simulink model "guidebot_mil"  (R2024a)
settings: Solver=FixedStepDiscrete  StartTime=0  StopTime=60.0  FixedStep=0.05  RelTol=1e-3
InitFcn:
  | gb_setup_base();
undefined symbols (not defined in the file or in its folder): GB_X0
settings Model: Creator=asus  LastModifiedBy=asus

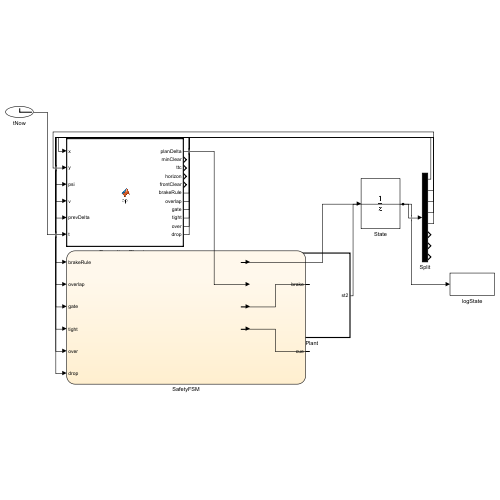
[thumbnail: Simulink's stored preview of the top-level diagram]
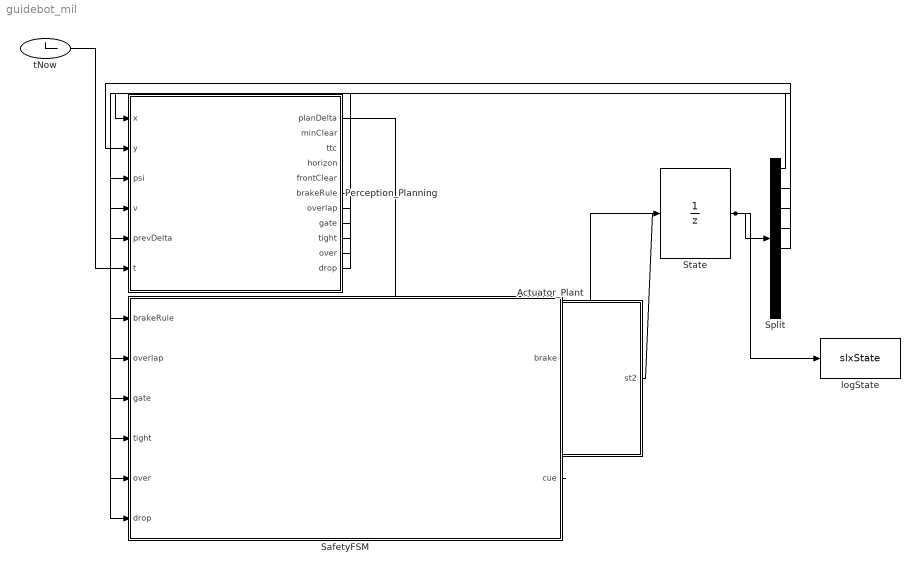
== system guidebot_mil ==
  Actuator_Plant : MATLAB Function  TreatAsAtomicUnit=on
  Perception_Planning : MATLAB Function  TreatAsAtomicUnit=on
  SafetyFSM : Stateflow chart  TreatAsAtomicUnit=on
  Split : Demux  Outputs=8
  State : UnitDelay  InitialCondition=GB_X0  SampleTime=0.05  HasFrameUpgradeWarning=on
  logState : ToWorkspace  VariableName=slxState  SaveFormat=Structure With Time  SampleTime=-1
  tNow : Clock
  wires:
  State/1 -> Split/1, Actuator_Plant/1(st), logState/1
  tNow/1 -> Perception_Planning/6(t)
  Split/1 -> Perception_Planning/1(x)
  Split/2 -> Perception_Planning/2(y)
  Split/3 -> Perception_Planning/3(psi)
  Split/4 -> Perception_Planning/4(v)
  Split/5 -> Perception_Planning/5(prevDelta)
  Perception_Planning/1(planDelta) -> Actuator_Plant/2(planDelta)
  Perception_Planning/6(brakeRule) -> SafetyFSM/1(brakeRule)
  Perception_Planning/7(overlap) -> SafetyFSM/2(overlap)
  Perception_Planning/8(gate) -> SafetyFSM/3(gate)
  Perception_Planning/9(tight) -> SafetyFSM/4(tight)
  Perception_Planning/10(over) -> SafetyFSM/5(over)
  Perception_Planning/11(drop) -> SafetyFSM/6(drop)
  SafetyFSM/1(brake) -> Actuator_Plant/3(brake)
  SafetyFSM/2(cue) -> Actuator_Plant/4(cue)
  Actuator_Plant/1(st2) -> State/1

== matlab function guidebot_mil/Actuator_Plant ==
  data: st input; st2 output; planDelta input; brake input; cue input
function st2 = ap(st,planDelta,brake,cue)
dt=0.050000; WB=0.450000; RR=0.220000; HW=2.000000;
pref=1.150000; slowF=0.500000; Tr=0.350000; slewDps=150.000000;
x=st(1); y=st(2); psi=st(3); v=st(4); prevDelta=st(5); tgt=st(6); bk=st(7); held=st(8);
maxStep=(slewDps*pi/180.0)*dt;
delta=planDelta; step=delta-prevDelta;
if step>maxStep, step=maxStep; end
if step<-maxStep, step=-maxStep; end
delta=prevDelta+step;
if brake>0, delta=prevDelta*0.5; end
if bk>0
    tgt=-0.30;
elseif abs(cue-4.0)<0.5
    tgt=0.0;
elseif abs(cue-3.0)<0.5
    tgt=pref*slowF;
else
    tgt=pref;
end
v = v + (tgt-v)*(dt/Tr);
if brake>0, v = v - 3.2*dt; end
v = max(-0.45, min(2.0, v));
if abs(v)>1e-4
    psi = psi + v*tan(delta)/WB*dt;
    x = x + v*cos(psi)*dt;
    y = y + v*sin(psi)*dt;
    lim = HW-RR;
    if abs(y)>lim, y = sign(y)*lim; psi = 0.0; end
end
if brake>0 && abs(v)<0.06, held = held + dt; else, held = 0.0; end
if held>5.0, bk = 1.2; held = 0.0; end
bk = max(0.0, bk-dt);
st2 = [x;y;psi;v;delta;tgt;bk;held];
end

== matlab function guidebot_mil/Perception_Planning ==
  data: x input; planDelta output; y input; psi input; v input; prevDelta input; t input; minClear output; ttc output; horizon output; frontClear output; brakeRule output; overlap output; gate output; tight output; over output; drop output
function [planDelta,minClear,ttc,horizon,frontClear,brakeRule,overlap,gate,tight,over,drop] = pp(x,y,psi,v,prevDelta,t)
coder.extrinsic('gb_ai_host_step');
planDelta=0; minClear=1e9; ttc=1e9; horizon=1.0; frontClear=1e9; over=false; drop=false;
[planDelta,minClear,ttc,horizon,frontClear,over,drop] = gb_ai_host_step(x,y,psi,v,prevDelta,t);
deltaMax=0.436332312999; wheelbase=0.450000000000; mu=0.600000000000; g=9.810000000000; latency=0.100000000000;
margin=0.120000000000; vMin=0.300000000000; bodyClear=0.150000000000; ttcBrakeS=0.900000000000; safetyClear=0.250000000000;
brakeRule=false; overlap=false; gate=false; tight=false; dReq=0; latCan=0; latNeed=0;
[b0,b1,b2,b3,dReq,latCan,latNeed] = gb_safety_compute(minClear,frontClear,ttc,v,horizon,deltaMax,wheelbase,mu,g,latency,margin,vMin,bodyClear,ttcBrakeS,safetyClear);
brakeRule=logical(b0); overlap=logical(b1); gate=logical(b2); tight=logical(b3);
end

== stateflow chart guidebot_mil/SafetyFSM ==
  state NOMINAL
    entry: brake=0; cue=0;
  state HAZARD_OVER
    entry: brake=0; cue=5;
  state STOP
    entry: brake=1; cue=4;
  state SLOW
    entry: brake=0; cue=3;
  state HAZARD_DROP
    entry: brake=0; cue=6;
  STOP -> NOMINAL : [~(brakeRule || overlap || gate)]
  HAZARD_OVER -> NOMINAL [order 2] : [~over]
  HAZARD_DROP -> NOMINAL [order 2] : [~drop]
  (default) -> NOMINAL
  SLOW -> NOMINAL [order 2] : [~tight]
  NOMINAL -> HAZARD_OVER [order 2] : [over]
  NOMINAL -> HAZARD_DROP [order 3] : [drop]
  NOMINAL -> SLOW [order 4] : [tight]
  NOMINAL -> STOP [order 1] : [brakeRule || overlap || gate]
  HAZARD_OVER -> STOP [order 1] : [brakeRule || overlap || gate]
  SLOW -> STOP [order 1] : [brakeRule || overlap || gate]
  HAZARD_DROP -> STOP [order 1] : [brakeRule || overlap || gate]
  data: brakeRule input; overlap input; gate input; tight input; over input; drop input; brake output; cue output
